simulink model "skarab_fgbe"  (R2018a)
settings: Solver=VariableStepDiscrete  StartTime=0.0  StopTime=50000  RelTol=1e-3
libraries: xbsIndex_r4 x704, casper_library_misc x5, xps_library x3
(part 1 of 9)
settings Model: Creator=cicada  LastModifiedBy=aisaacson
settings SolverCC: ZeroCrossControl=EnableAll
settings DataIOCC: LimitDataPoints=on  SaveFormat=Array  SignalLoggingSaveFormat=ModelDataLogs
settings OptimizationCC: DefaultParameterBehavior=Inlined  ExpressionDepthLimit=2147483647  LifeSpan=inf
settings DebuggingCC: WriteAfterWriteMsg=EnableAllAsError  SignalResolutionControl=TryResolveAllWithWarning  SolverPrmCheckMsg=warning  FcnCallInpInsideContextMsg=warning  AllowSymbolicDim=off  StateNameClashWarn=warning  LibraryContextMissingDiagnostic=warning  StrictBusMsg=ErrorOnBusTreatedAsVector  SFUnexpectedBacktrackingDiag=warning  SFNoUnconditionalDefaultTransitionDiag=warning  SFExecutionAtInitializationDiag=none
settings HardwareCC: ProdBitPerPointer=32  ProdBitPerSizeT=32  ProdBitPerPtrDiffT=32  ProdLargestAtomicFloat=None  ProdIntDivRoundTo=Undefined  ProdEndianess=Unspecified  ProdWordSize=32  ProdHWDeviceType=32-bit Generic
settings ModelReferenceCC: PropagateSignalLabelsOutOfModel=off
settings CodeAppCC: StateflowObjectComments=on
settings GRTTargetCC: TargetLangStandard=C89/C90 (ANSI)  GeneratePreprocessorConditionals=Disable all  CombineOutputUpdateFcns=off  GRTInterface=on
settings ConfigComp: CovMetricSettings=dw  CovHtmlReporting=on  CovSaveCumulativeToWorkspaceVar=on  CovSaveSingleToWorkspaceVar=on  CovExternalEMLEnable=off

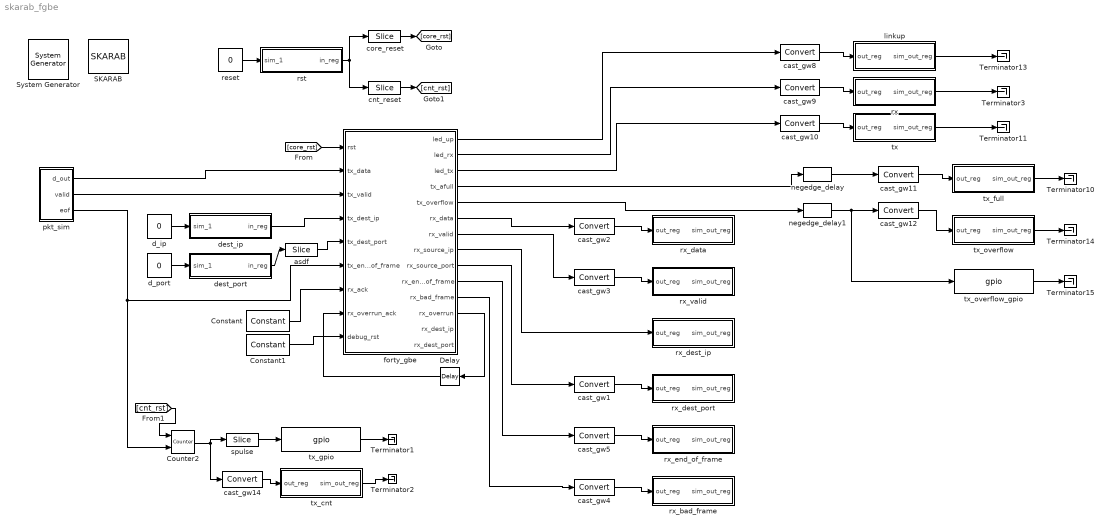
== system skarab_fgbe ==
  " System Generator" : xbsIndex_r4/ System Generator  Tag=genX  xilinxfamily=virtex7  part=xc7vx690t  speed=-2  package=ffg1927  synthesis_tool=XST  clock_wrapper=Clock Enables  directory=/data/casper/mlib_devel_sw_reg_defaults/jasper_library/test_models/skarab_fgbe/sysgen  proj_type=Project Navigator  Synth_file=XST Defaults  Impl_file=ISE Defaults  testbench=off  simulink_period=1  sysclk_period=5.8824  dcm_input_clock_period=10  incr_netlist=off  trim_vbits=Everywhere in SubSystem  dbl_ovrd=According to Block Masks  core_generation=According to Block Masks  run_coregen=off  deprecated_control=off  eval_field=0  block_type=sysgen
      settings: block_version=11.4
  Constant : xbsIndex_r4/Constant  const=1  gui_display_data_type=Boolean  arith_type=Boolean  n_bits=16  bin_pt=14  preci_type=Single  exp_width=8  frac_width=24  explicit_period=on  period=1  equ=P=C  opselect=C  inp2=PCIN>>17  opr=+  inp1=P  carry=CIN  dbl_ovrd=off  block_type=constant
  Constant1 : xbsIndex_r4/Constant  const=0  gui_display_data_type=Boolean  arith_type=Boolean  n_bits=16  bin_pt=14  preci_type=Single  exp_width=8  frac_width=24  explicit_period=on  period=1  equ=P=C  opselect=C  inp2=PCIN>>17  opr=+  inp1=P  carry=CIN  dbl_ovrd=off  block_type=constant
  Counter2 : xbsIndex_r4/Counter  cnt_type=Free Running  cnt_to=Inf  operation=Up  start_count=0  cnt_by_val=1  arith_type=Unsigned  n_bits=32  bin_pt=0  load_pin=off  rst=on  en=on  explicit_period=on  period=1  use_behavioral_HDL=off  implementation=Fabric  dbl_ovrd=off  block_type=counter
      settings: block_version=11.4
  Delay : xbsIndex_r4/Delay  rst=off  infoeditControl=Selection of Reset will increase slice count due to use of real FFs and instead of SRLs  en=off  latency=1  reg_retiming=on  dbl_ovrd=off  block_type=delay
      settings: block_version=11.4
  SKARAB : xps_library/Platforms/SKARAB  Tag=xps:xsg  hw_sys=SKARAB:xc7vx690t  clk_src=sys_clk  clk_rate=170  sample_period=1  synthesis_tool=XST
      settings: SourceProductName=CASPER XPS Blockset
  Terminator{1..3,10..11,13..15} (8 alike) : Terminator
  asdf : xbsIndex_r4/Slice  nbits=16  boolean_output=off  mode=Lower Bit Location + Width  bit1=0  base1=MSB of Input  bit0=0  base0=LSB of Input  dbl_ovrd=off  block_type=slice
  cast_gw{1..5,8..12,14} (11 alike) : xbsIndex_r4/Convert  gui_display_data_type=Fixed-point  arith_type=Unsigned  n_bits=32  bin_pt=0  float_type=Single  exp_bits=8  fraction_bits=24  quantization=Truncate  overflow=Wrap  en=off  latency=0  pipeline=off  dbl_ovrd=off  block_type=convert
  cnt_reset : xbsIndex_r4/Slice  nbits=1  boolean_output=on  mode=Lower Bit Location + Width  bit1=0  base1=MSB of Input  bit0=0  base0=LSB of Input  dbl_ovrd=off  block_type=slice
  core_reset : xbsIndex_r4/Slice  nbits=1  boolean_output=on  mode=Lower Bit Location + Width  bit1=0  base1=MSB of Input  bit0=1  base0=LSB of Input  dbl_ovrd=off  block_type=slice
  d_ip : Constant  Value=0
  d_port : Constant  Value=0
  dest_ip : Subsystem  Tag=xps:sw_reg  AncestorBlock=xps_library/Memory/software_register  mask(swreg){io_dir=From Processor, io_delay=0, init_val=1234, sample_period=1, names=reg, bitwidths=32, bin_pts=0, arith_types=0, sim_port=on, show_format=on}
      mask prompts: io_dir "I/O direction"; io_delay "I/O delay"; init_val "Initial Value"; sample_period "Sample period"; names "Bitfield names [msb...lsb]"; bitwidths "Bitfield widths"; bin_pts "Bitfield binary pts"; arith_types "Bitfield types, ufix=0, fix=1, bool=2"; sim_port "Provide sim input/output?"; show_format "Print format string?"
      mask help: A 32-bit software-accessible register. Can be divided into bitfields of varying widths and types using the fields in the block mask.
      mask init:
      | swreg_init(gcb)
      settings: AttributesFormatString=1input:uf32.0 = 32 bits
      mask TypeOptions io_dir: To Processor | From Processor
      mask Callback io_dir:
      | mask_enables = get_param(gcb, 'MaskEnables');
      | mask_names = get_param(gcb, 'MaskNames');
      | if strcmp(get_param(gcb, 'io_dir'), 'To Processor'),
      |     mask_enables{ismember(mask_names, 'sample_period')} = 'off';
      | else
      |     mask_enables{ismember(mask_names, 'sample_period')} = 'on';
      | end
      | set_param(gcb, 'MaskEnables', mask_enables);
      mask DialogControl ParameterTabVar0 Prompt: Setup
  dest_port : Subsystem  Tag=xps:sw_reg  AncestorBlock=xps_library/Memory/software_register  mask(swreg){io_dir=From Processor, io_delay=0, init_val=64000, sample_period=1, names=reg, bitwidths=32, bin_pts=0, arith_types=0, sim_port=on, show_format=on}
      mask prompts: io_dir "I/O direction"; io_delay "I/O delay"; init_val "Initial Value"; sample_period "Sample period"; names "Bitfield names [msb...lsb]"; bitwidths "Bitfield widths"; bin_pts "Bitfield binary pts"; arith_types "Bitfield types, ufix=0, fix=1, bool=2"; sim_port "Provide sim input/output?"; show_format "Print format string?"
      mask help: A 32-bit software-accessible register. Can be divided into bitfields of varying widths and types using the fields in the block mask.
      mask init:
      | swreg_init(gcb)
      settings: AttributesFormatString=1input:uf32.0 = 32 bits
      mask TypeOptions io_dir: To Processor | From Processor
      mask Callback io_dir:
      | mask_enables = get_param(gcb, 'MaskEnables');
      | mask_names = get_param(gcb, 'MaskNames');
      | if strcmp(get_param(gcb, 'io_dir'), 'To Processor'),
      |     mask_enables{ismember(mask_names, 'sample_period')} = 'off';
      | else
      |     mask_enables{ismember(mask_names, 'sample_period')} = 'on';
      | end
      | set_param(gcb, 'MaskEnables', mask_enables);
      mask DialogControl ParameterTabVar0 Prompt: Setup
  forty_gbe : Subsystem  Tag=xps:forty_gbe  AncestorBlock=xps_library/IO/forty_gbe  mask(forty_gbe){flavour=cx4, slot=1, port_r1=0, port_r2_cx4=0, port_r2_sfpp=0, port=0, rx_dist_ram=on, large_frames=off, input_pipeline_delay=3, show_param=off, pre_emph_r2=0.74, pre_emph=3, post_emph_r2=0.18, rxeqmix_r2=7, swing_r2=940, swing=800, fab_en=on, fab_mac=hex2dec('123456780000'), fab_ip=192*(2^24) + 168*(2^16) + 5*(2^8) + 20*(2^0), fab_udp=10000, fab_gate=1, cpu_rx_en=on, cpu_tx_en=on, ttl=hex2dec('FF'), promisc_mode=off, debug_ctr_width=16, debug_en_all=off, debug_dis_all=off, txctr=off, txerrctr=off, txerrctr_len=100, txofctr=off, txfullctr=off, txvldctr=off, txsnaplen=256, rxctr=off, rxerrctr=off, rxerrctr_len=100, rxofctr=off, rxbadctr=off, rxvldctr=off, rxeofctr=off, rxsnaplen=0 - no snap, rxsrcip=on, rxdstip=on}
      mask prompts: flavour "Mezzanine card flavour"; slot "Card slot"; port_r1 "Port"; port_r2_cx4 "Port"; port_r2_sfpp "Port"; rx_dist_ram "Shallow RX Fifo (Beware overruns!)"; large_frames "Enable Large TX Frames (8k+512)"; input_pipeline_delay "Incoming pipeline delay"; show_param "---------------------- Show Implementation Parameters -----------------------------------------------------------------------------------"; pre_emph_r2 "Pre-emphasis (dB)"; pre_emph "Pre-emphasis"; post_emph_r2 "Post-emphasis (dB)"; rxeqmix_r2 "Receive equalisation"; swing_r2 "Driver Swing Control (mVppd)"; swing "Differential swing"; fab_en "Enable fabric on startup"; fab_mac "Fabric MAC Address"; fab_ip "Fabric IP Address"; fab_udp "Fabric UDP Port"; fab_gate "Fabric Gateway"; cpu_rx_en "Enable CPU RX"; cpu_tx_en "Enable CPU TX"; promisc_mode "Promiscuous mode"; debug_ctr_width "Debug counter width"; debug_en_all "Enable all counters (overrides individual settings)"; debug_dis_all "Disable all counters (overrides individual settings)"; txctr "TX - core_txctr"; txerrctr "TX packet length error - core_txerrctr"; txerrctr_len "-- expected TX packet length"; txofctr "TX overflow - core_txofctr"; txfullctr "TX full - core_txfullctr"; txvldctr "TX valid cycle - core_txvldctr"; txsnaplen "TX snapshot length"; rxctr "RX - core_rxctr"; rxerrctr "RX packet length error - core_rxerrctr"; rxerrctr_len "-- expected RX packet length"; rxofctr "RX overflow - core_rxofctr"; rxbadctr "RX bad - core_rxbadctr"; rxvldctr "RX valid cycle - core_rxvldctr"; rxeofctr "RX eof - core_rxeofctr"; rxsnaplen "RX snapshot length"; rxsrcip "RX snapshot - include source IPs"; rxdstip "RX snapshot - include destination IPs"
      mask help: This block sends and receives UDP frames (packets). It accepts a 64 bit wide data stream with user-determined frame breaks. The data stream is wrapped in a UDP frame for transmission. Incoming UDP packets are unwrapped and the data presented as a 64 bit wide stream.
      mask init:
      | temp = eval(get_param(gcb, 'debug_ctr_width'));
      | if temp <= 0,
      |     error('Debug counters cannot be <= zero.');
      | end
      | forty_gbe_mask(gcb)
      settings: AttributesFormatString=incoming_latency=3
      mask TypeOptions flavour: sfp+ | cx4
      mask Callback flavour: forty_gbe_callback
      mask TypeOptions slot: 0 | 1
      mask TypeOptions port_r1: 0 | 1 | 2 | 3
      mask TypeOptions port_r2_cx4: 0 | 1 | 2
      mask TypeOptions port_r2_sfpp: 0 | 1 | 2 | 3
      mask TypeOptions port: 0 | 1 | 2 | 3
      mask Callback show_param: forty_gbe_callback
      mask TypeOptions pre_emph_r2: 0.15 | 0.3 | 0.45 | 0.61 | 0.74 | 0.91 | 1.07 | 1.25 | 1.36 | 1.55 | 1.74 | 1.94 | 2.11 | 2.32 | 2.54 | 2.77
      mask TypeOptions pre_emph: 0 | 1 | 2 | 3
      mask TypeOptions post_emph_r2: 0.18 | 0.19 | 0.2 | 0.39 | 0.63 | 0.82 | 1.07 | 1.32 | 1.6 | 1.65 | 1.94 | 2.21 | 2.52 | 2.76 | 3.08 | 3.41 | 3.77 | 3.97 | 4.36 | 4.73 | 5.16 | 5.47 | 5.93 | 6.38 | 6.89
      mask TypeOptions rxeqmix_r2: 0 | 1 | 2 | 3 | 4 | 5 | 6 | 7
      mask TypeOptions swing_r2: 110 | 210 | 310 | 400 | 480 | 570 | 660 | 740 | 810 | 880 | 940 | 990 | 1040 | 1080 | 1110 | 1130
      mask TypeOptions swing: 400 | 500 | 600 | 700 | 800
      mask Callback debug_en_all:
      | if strcmp(get_param(gcb, 'debug_en_all'), 'on')
      |     set_param(gcb, 'debug_dis_all', 'off')
      | end
      mask Callback debug_dis_all:
      | if strcmp(get_param(gcb, 'debug_dis_all'), 'on')
      |     set_param(gcb, 'debug_en_all', 'off')
      | end
      mask Callback txerrctr:
      | blk = gcb;
      | mask_visibilities = get_param(blk, 'MaskVisibilities');
      | mask_names = get_param(blk, 'MaskNames');
      | if strcmp(get_param(blk, 'txerrctr'), 'on')
      |     mask_visibilities{ismember(mask_names, 'txerrctr_len')} = 'on';
      | else
      |     mask_visibilities{ismember(mask_names, 'txerrctr_len')} = 'off';
      | end
      | set_param(blk, 'MaskVisibilities', mask_visibilities);
      mask TypeOptions txsnaplen: 0 - no snap | 256 | 512 | 1024 | 2048 | 4096 | 8192 | 16384
      mask Callback rxerrctr:
      | blk = gcb;
      | mask_visibilities = get_param(blk, 'MaskVisibilities');
      | mask_names = get_param(blk, 'MaskNames');
      | if strcmp(get_param(blk, 'rxerrctr'), 'on')
      |     mask_visibilities{ismember(mask_names, 'rxerrctr_len')} = 'on';
      | else
      |     mask_visibilities{ismember(mask_names, 'rxerrctr_len')} = 'off';
      | end
      | set_param(blk, 'MaskVisibilities', mask_visibilities);
      mask TypeOptions rxsnaplen: 0 - no snap | 256 | 512 | 1024 | 2048 | 4096 | 8192 | 16384
      mask DialogControl ParameterTabVar0 Prompt: Core
      mask DialogControl ParameterTabVar01 Prompt: Debug counters
      mask DialogControl Control2 Prompt: -------------------------------------
      mask DialogControl Control2_copy Prompt: -------------------------------------
  linkup : Subsystem  Tag=xps:sw_reg  AncestorBlock=xps_library/Memory/software_register  mask(swreg){io_dir=To Processor, io_delay=0, init_val=0, sample_period=1, names=reg, bitwidths=32, bin_pts=0, arith_types=0, sim_port=on, show_format=on}
      mask prompts: io_dir "I/O direction"; io_delay "I/O delay"; init_val "Initial Value"; sample_period "Sample period"; names "Bitfield names [msb...lsb]"; bitwidths "Bitfield widths"; bin_pts "Bitfield binary pts"; arith_types "Bitfield types, ufix=0, fix=1, bool=2"; sim_port "Provide sim input/output?"; show_format "Print format string?"
      mask help: A 32-bit software-accessible register. Can be divided into bitfields of varying widths and types using the fields in the block mask.
      mask init:
      | swreg_init(gcb)
      settings: AttributesFormatString=1output:uf32.0 = 32 bits
      mask TypeOptions io_dir: To Processor | From Processor
      mask Callback io_dir:
      | mask_enables = get_param(gcb, 'MaskEnables');
      | mask_names = get_param(gcb, 'MaskNames');
      | if strcmp(get_param(gcb, 'io_dir'), 'To Processor'),
      |     mask_enables{ismember(mask_names, 'sample_period')} = 'off';
      | else
      |     mask_enables{ismember(mask_names, 'sample_period')} = 'on';
      | end
      | set_param(gcb, 'MaskEnables', mask_enables);
      mask DialogControl ParameterTabVar0 Prompt: Setup
  negedge_delay : casper_library_misc/negedge_delay  pulse_len=2^20
      settings: SourceProductName=CASPER DSP Blockset
  negedge_delay1 : casper_library_misc/negedge_delay  pulse_len=2^20
      settings: SourceProductName=CASPER DSP Blockset
  pkt_sim : Subsystem
  reset : Constant  Value=0
  rst : Subsystem  Tag=xps:sw_reg  AncestorBlock=xps_library/Memory/software_register  mask(swreg){io_dir=From Processor, io_delay=0, init_val=0, sample_period=1, names=reg, bitwidths=32, bin_pts=0, arith_types=0, sim_port=on, show_format=on}
      mask prompts: io_dir "I/O direction"; io_delay "I/O delay"; init_val "Initial Value"; sample_period "Sample period"; names "Bitfield names [msb...lsb]"; bitwidths "Bitfield widths"; bin_pts "Bitfield binary pts"; arith_types "Bitfield types, ufix=0, fix=1, bool=2"; sim_port "Provide sim input/output?"; show_format "Print format string?"
      mask help: A 32-bit software-accessible register. Can be divided into bitfields of varying widths and types using the fields in the block mask.
      mask init:
      | swreg_init(gcb)
      settings: AttributesFormatString=1input:uf32.0 = 32 bits
      mask TypeOptions io_dir: To Processor | From Processor
      mask Callback io_dir:
      | mask_enables = get_param(gcb, 'MaskEnables');
      | mask_names = get_param(gcb, 'MaskNames');
      | if strcmp(get_param(gcb, 'io_dir'), 'To Processor'),
      |     mask_enables{ismember(mask_names, 'sample_period')} = 'off';
      | else
      |     mask_enables{ismember(mask_names, 'sample_period')} = 'on';
      | end
      | set_param(gcb, 'MaskEnables', mask_enables);
      mask DialogControl ParameterTabVar0 Prompt: Setup
  rx : Subsystem  Tag=xps:sw_reg  AncestorBlock=xps_library/Memory/software_register  mask(swreg){io_dir=To Processor, io_delay=0, init_val=0, sample_period=1, names=reg, bitwidths=32, bin_pts=0, arith_types=0, sim_port=on, show_format=on}
      mask prompts: io_dir "I/O direction"; io_delay "I/O delay"; init_val "Initial Value"; sample_period "Sample period"; names "Bitfield names [msb...lsb]"; bitwidths "Bitfield widths"; bin_pts "Bitfield binary pts"; arith_types "Bitfield types, ufix=0, fix=1, bool=2"; sim_port "Provide sim input/output?"; show_format "Print format string?"
      mask help: A 32-bit software-accessible register. Can be divided into bitfields of varying widths and types using the fields in the block mask.
      mask init:
      | swreg_init(gcb)
      settings: AttributesFormatString=1output:uf32.0 = 32 bits
      mask TypeOptions io_dir: To Processor | From Processor
      mask Callback io_dir:
      | mask_enables = get_param(gcb, 'MaskEnables');
      | mask_names = get_param(gcb, 'MaskNames');
      | if strcmp(get_param(gcb, 'io_dir'), 'To Processor'),
      |     mask_enables{ismember(mask_names, 'sample_period')} = 'off';
      | else
      |     mask_enables{ismember(mask_names, 'sample_period')} = 'on';
      | end
      | set_param(gcb, 'MaskEnables', mask_enables);
      mask DialogControl ParameterTabVar0 Prompt: Setup
  rx_bad_frame : Subsystem  Tag=xps:sw_reg  AncestorBlock=xps_library/Memory/software_register  mask(swreg){io_dir=To Processor, io_delay=0, init_val=0, sample_period=1, names=reg, bitwidths=32, bin_pts=0, arith_types=0, sim_port=on, show_format=on}
      mask prompts: io_dir "I/O direction"; io_delay "I/O delay"; init_val "Initial Value"; sample_period "Sample period"; names "Bitfield names [msb...lsb]"; bitwidths "Bitfield widths"; bin_pts "Bitfield binary pts"; arith_types "Bitfield types, ufix=0, fix=1, bool=2"; sim_port "Provide sim input/output?"; show_format "Print format string?"
      mask help: A 32-bit software-accessible register. Can be divided into bitfields of varying widths and types using the fields in the block mask.
      mask init:
      | swreg_init(gcb)
      settings: AttributesFormatString=1output:uf32.0 = 32 bits
      mask TypeOptions io_dir: To Processor | From Processor
      mask Callback io_dir:
      | mask_enables = get_param(gcb, 'MaskEnables');
      | mask_names = get_param(gcb, 'MaskNames');
      | if strcmp(get_param(gcb, 'io_dir'), 'To Processor'),
      |     mask_enables{ismember(mask_names, 'sample_period')} = 'off';
      | else
      |     mask_enables{ismember(mask_names, 'sample_period')} = 'on';
      | end
      | set_param(gcb, 'MaskEnables', mask_enables);
      mask DialogControl ParameterTabVar0 Prompt: Setup
  rx_data : Subsystem  Tag=xps:sw_reg  AncestorBlock=xps_library/Memory/software_register  mask(swreg){io_dir=To Processor, io_delay=0, init_val=0, sample_period=1, names=reg, bitwidths=32, bin_pts=0, arith_types=0, sim_port=on, show_format=on}
      mask prompts: io_dir "I/O direction"; io_delay "I/O delay"; init_val "Initial Value"; sample_period "Sample period"; names "Bitfield names [msb...lsb]"; bitwidths "Bitfield widths"; bin_pts "Bitfield binary pts"; arith_types "Bitfield types, ufix=0, fix=1, bool=2"; sim_port "Provide sim input/output?"; show_format "Print format string?"
      mask help: A 32-bit software-accessible register. Can be divided into bitfields of varying widths and types using the fields in the block mask.
      mask init:
      | swreg_init(gcb)
      settings: AttributesFormatString=1output:uf32.0 = 32 bits
      mask TypeOptions io_dir: To Processor | From Processor
      mask Callback io_dir:
      | mask_enables = get_param(gcb, 'MaskEnables');
      | mask_names = get_param(gcb, 'MaskNames');
      | if strcmp(get_param(gcb, 'io_dir'), 'To Processor'),
      |     mask_enables{ismember(mask_names, 'sample_period')} = 'off';
      | else
      |     mask_enables{ismember(mask_names, 'sample_period')} = 'on';
      | end
      | set_param(gcb, 'MaskEnables', mask_enables);
      mask DialogControl ParameterTabVar0 Prompt: Setup
  rx_dest_ip : Subsystem  Tag=xps:sw_reg  AncestorBlock=xps_library/Memory/software_register  mask(swreg){io_dir=To Processor, io_delay=0, init_val=0, sample_period=1, names=reg, bitwidths=32, bin_pts=0, arith_types=0, sim_port=on, show_format=on}
      mask prompts: io_dir "I/O direction"; io_delay "I/O delay"; init_val "Initial Value"; sample_period "Sample period"; names "Bitfield names [msb...lsb]"; bitwidths "Bitfield widths"; bin_pts "Bitfield binary pts"; arith_types "Bitfield types, ufix=0, fix=1, bool=2"; sim_port "Provide sim input/output?"; show_format "Print format string?"
      mask help: A 32-bit software-accessible register. Can be divided into bitfields of varying widths and types using the fields in the block mask.
      mask init:
      | swreg_init(gcb)
      settings: AttributesFormatString=1output:uf32.0 = 32 bits
      mask TypeOptions io_dir: To Processor | From Processor
      mask Callback io_dir:
      | mask_enables = get_param(gcb, 'MaskEnables');
      | mask_names = get_param(gcb, 'MaskNames');
      | if strcmp(get_param(gcb, 'io_dir'), 'To Processor'),
      |     mask_enables{ismember(mask_names, 'sample_period')} = 'off';
      | else
      |     mask_enables{ismember(mask_names, 'sample_period')} = 'on';
      | end
      | set_param(gcb, 'MaskEnables', mask_enables);
      mask DialogControl ParameterTabVar0 Prompt: Setup
  rx_dest_port : Subsystem  Tag=xps:sw_reg  AncestorBlock=xps_library/Memory/software_register  mask(swreg){io_dir=To Processor, io_delay=0, init_val=0, sample_period=1, names=reg, bitwidths=32, bin_pts=0, arith_types=0, sim_port=on, show_format=on}
      mask prompts: io_dir "I/O direction"; io_delay "I/O delay"; init_val "Initial Value"; sample_period "Sample period"; names "Bitfield names [msb...lsb]"; bitwidths "Bitfield widths"; bin_pts "Bitfield binary pts"; arith_types "Bitfield types, ufix=0, fix=1, bool=2"; sim_port "Provide sim input/output?"; show_format "Print format string?"
      mask help: A 32-bit software-accessible register. Can be divided into bitfields of varying widths and types using the fields in the block mask.
      mask init:
      | swreg_init(gcb)
      settings: AttributesFormatString=1output:uf32.0 = 32 bits
      mask TypeOptions io_dir: To Processor | From Processor
      mask Callback io_dir:
      | mask_enables = get_param(gcb, 'MaskEnables');
      | mask_names = get_param(gcb, 'MaskNames');
      | if strcmp(get_param(gcb, 'io_dir'), 'To Processor'),
      |     mask_enables{ismember(mask_names, 'sample_period')} = 'off';
      | else
      |     mask_enables{ismember(mask_names, 'sample_period')} = 'on';
      | end
      | set_param(gcb, 'MaskEnables', mask_enables);
      mask DialogControl ParameterTabVar0 Prompt: Setup
  rx_end_of_frame : Subsystem  Tag=xps:sw_reg  AncestorBlock=xps_library/Memory/software_register  mask(swreg){io_dir=To Processor, io_delay=0, init_val=0, sample_period=1, names=reg, bitwidths=32, bin_pts=0, arith_types=0, sim_port=on, show_format=on}
      mask prompts: io_dir "I/O direction"; io_delay "I/O delay"; init_val "Initial Value"; sample_period "Sample period"; names "Bitfield names [msb...lsb]"; bitwidths "Bitfield widths"; bin_pts "Bitfield binary pts"; arith_types "Bitfield types, ufix=0, fix=1, bool=2"; sim_port "Provide sim input/output?"; show_format "Print format string?"
      mask help: A 32-bit software-accessible register. Can be divided into bitfields of varying widths and types using the fields in the block mask.
      mask init:
      | swreg_init(gcb)
      settings: AttributesFormatString=1output:uf32.0 = 32 bits
      mask TypeOptions io_dir: To Processor | From Processor
      mask Callback io_dir:
      | mask_enables = get_param(gcb, 'MaskEnables');
      | mask_names = get_param(gcb, 'MaskNames');
      | if strcmp(get_param(gcb, 'io_dir'), 'To Processor'),
      |     mask_enables{ismember(mask_names, 'sample_period')} = 'off';
      | else
      |     mask_enables{ismember(mask_names, 'sample_period')} = 'on';
      | end
      | set_param(gcb, 'MaskEnables', mask_enables);
      mask DialogControl ParameterTabVar0 Prompt: Setup
  rx_valid : Subsystem  Tag=xps:sw_reg  AncestorBlock=xps_library/Memory/software_register  mask(swreg){io_dir=To Processor, io_delay=0, init_val=0, sample_period=1, names=reg, bitwidths=32, bin_pts=0, arith_types=0, sim_port=on, show_format=on}
      mask prompts: io_dir "I/O direction"; io_delay "I/O delay"; init_val "Initial Value"; sample_period "Sample period"; names "Bitfield names [msb...lsb]"; bitwidths "Bitfield widths"; bin_pts "Bitfield binary pts"; arith_types "Bitfield types, ufix=0, fix=1, bool=2"; sim_port "Provide sim input/output?"; show_format "Print format string?"
      mask help: A 32-bit software-accessible register. Can be divided into bitfields of varying widths and types using the fields in the block mask.
      mask init:
      | swreg_init(gcb)
      settings: AttributesFormatString=1output:uf32.0 = 32 bits
      mask TypeOptions io_dir: To Processor | From Processor
      mask Callback io_dir:
      | mask_enables = get_param(gcb, 'MaskEnables');
      | mask_names = get_param(gcb, 'MaskNames');
      | if strcmp(get_param(gcb, 'io_dir'), 'To Processor'),
      |     mask_enables{ismember(mask_names, 'sample_period')} = 'off';
      | else
      |     mask_enables{ismember(mask_names, 'sample_period')} = 'on';
      | end
      | set_param(gcb, 'MaskEnables', mask_enables);
      mask DialogControl ParameterTabVar0 Prompt: Setup
  spulse : xbsIndex_r4/Slice  nbits=1  boolean_output=on  mode=Lower Bit Location + Width  bit1=0  base1=MSB of Input  bit0=27-12  base0=LSB of Input  dbl_ovrd=off  block_type=slice
  tx : Subsystem  Tag=xps:sw_reg  AncestorBlock=xps_library/Memory/software_register  mask(swreg){io_dir=To Processor, io_delay=0, init_val=0, sample_period=1, names=reg, bitwidths=32, bin_pts=0, arith_types=0, sim_port=on, show_format=on}
      mask prompts: io_dir "I/O direction"; io_delay "I/O delay"; init_val "Initial Value"; sample_period "Sample period"; names "Bitfield names [msb...lsb]"; bitwidths "Bitfield widths"; bin_pts "Bitfield binary pts"; arith_types "Bitfield types, ufix=0, fix=1, bool=2"; sim_port "Provide sim input/output?"; show_format "Print format string?"
      mask help: A 32-bit software-accessible register. Can be divided into bitfields of varying widths and types using the fields in the block mask.
      mask init:
      | swreg_init(gcb)
      settings: AttributesFormatString=1output:uf32.0 = 32 bits
      mask TypeOptions io_dir: To Processor | From Processor
      mask Callback io_dir:
      | mask_enables = get_param(gcb, 'MaskEnables');
      | mask_names = get_param(gcb, 'MaskNames');
      | if strcmp(get_param(gcb, 'io_dir'), 'To Processor'),
      |     mask_enables{ismember(mask_names, 'sample_period')} = 'off';
      | else
      |     mask_enables{ismember(mask_names, 'sample_period')} = 'on';
      | end
      | set_param(gcb, 'MaskEnables', mask_enables);
      mask DialogControl ParameterTabVar0 Prompt: Setup
  tx_cnt : Subsystem  Tag=xps:sw_reg  AncestorBlock=xps_library/Memory/software_register  mask(swreg){io_dir=To Processor, io_delay=0, init_val=0, sample_period=1, names=reg, bitwidths=32, bin_pts=0, arith_types=0, sim_port=on, show_format=on}
      mask prompts: io_dir "I/O direction"; io_delay "I/O delay"; init_val "Initial Value"; sample_period "Sample period"; names "Bitfield names [msb...lsb]"; bitwidths "Bitfield widths"; bin_pts "Bitfield binary pts"; arith_types "Bitfield types, ufix=0, fix=1, bool=2"; sim_port "Provide sim input/output?"; show_format "Print format string?"
      mask help: A 32-bit software-accessible register. Can be divided into bitfields of varying widths and types using the fields in the block mask.
      mask init:
      | swreg_init(gcb)
      settings: AttributesFormatString=1output:uf32.0 = 32 bits
      mask TypeOptions io_dir: To Processor | From Processor
      mask Callback io_dir:
      | mask_enables = get_param(gcb, 'MaskEnables');
      | mask_names = get_param(gcb, 'MaskNames');
      | if strcmp(get_param(gcb, 'io_dir'), 'To Processor'),
      |     mask_enables{ismember(mask_names, 'sample_period')} = 'off';
      | else
      |     mask_enables{ismember(mask_names, 'sample_period')} = 'on';
      | end
      | set_param(gcb, 'MaskEnables', mask_enables);
      mask DialogControl ParameterTabVar0 Prompt: Setup
  tx_full : Subsystem  Tag=xps:sw_reg  AncestorBlock=xps_library/Memory/software_register  mask(swreg){io_dir=To Processor, io_delay=0, init_val=0, sample_period=1, names=reg, bitwidths=32, bin_pts=0, arith_types=0, sim_port=on, show_format=on}
      mask prompts: io_dir "I/O direction"; io_delay "I/O delay"; init_val "Initial Value"; sample_period "Sample period"; names "Bitfield names [msb...lsb]"; bitwidths "Bitfield widths"; bin_pts "Bitfield binary pts"; arith_types "Bitfield types, ufix=0, fix=1, bool=2"; sim_port "Provide sim input/output?"; show_format "Print format string?"
      mask help: A 32-bit software-accessible register. Can be divided into bitfields of varying widths and types using the fields in the block mask.
      mask init:
      | swreg_init(gcb)
      settings: AttributesFormatString=1output:uf32.0 = 32 bits
      mask TypeOptions io_dir: To Processor | From Processor
      mask Callback io_dir:
      | mask_enables = get_param(gcb, 'MaskEnables');
      | mask_names = get_param(gcb, 'MaskNames');
      | if strcmp(get_param(gcb, 'io_dir'), 'To Processor'),
      |     mask_enables{ismember(mask_names, 'sample_period')} = 'off';
      | else
      |     mask_enables{ismember(mask_names, 'sample_period')} = 'on';
      | end
      | set_param(gcb, 'MaskEnables', mask_enables);
      mask DialogControl ParameterTabVar0 Prompt: Setup
  tx_gpio : xps_library/IO/gpio  Tag=xps:gpio  io_group_params_forwarded=on  io_group=ROACH:led  io_group_real=led  io_group_custom=0  io_dir=out  arith_type=Boolean  bitwidth=1  bin_pt=0  bit_index=0  sample_period=1  use_single_ended=off  use_ddr=off  reg_iob=on  reg_clk_phase=0  termination=None
      settings: SourceProductName=CASPER XPS Blockset
  tx_overflow : Subsystem  Tag=xps:sw_reg  AncestorBlock=xps_library/Memory/software_register  mask(swreg){io_dir=To Processor, io_delay=0, init_val=0, sample_period=1, names=reg, bitwidths=32, bin_pts=0, arith_types=0, sim_port=on, show_format=on}
      mask prompts: io_dir "I/O direction"; io_delay "I/O delay"; init_val "Initial Value"; sample_period "Sample period"; names "Bitfield names [msb...lsb]"; bitwidths "Bitfield widths"; bin_pts "Bitfield binary pts"; arith_types "Bitfield types, ufix=0, fix=1, bool=2"; sim_port "Provide sim input/output?"; show_format "Print format string?"
      mask help: A 32-bit software-accessible register. Can be divided into bitfields of varying widths and types using the fields in the block mask.
      mask init:
      | swreg_init(gcb)
      settings: AttributesFormatString=1output:uf32.0 = 32 bits
      mask TypeOptions io_dir: To Processor | From Processor
      mask Callback io_dir:
      | mask_enables = get_param(gcb, 'MaskEnables');
      | mask_names = get_param(gcb, 'MaskNames');
      | if strcmp(get_param(gcb, 'io_dir'), 'To Processor'),
      |     mask_enables{ismember(mask_names, 'sample_period')} = 'off';
      | else
      |     mask_enables{ismember(mask_names, 'sample_period')} = 'on';
      | end
      | set_param(gcb, 'MaskEnables', mask_enables);
      mask DialogControl ParameterTabVar0 Prompt: Setup
  tx_overflow_gpio : xps_library/IO/gpio  Tag=xps:gpio  io_group_params_forwarded=on  io_group=ROACH:led  io_group_real=led  io_group_custom=0  io_dir=out  arith_type=Boolean  bitwidth=1  bin_pt=0  bit_index=1  sample_period=1  use_single_ended=off  use_ddr=off  reg_iob=on  reg_clk_phase=0  termination=None
      settings: SourceProductName=CASPER XPS Blockset
  wires:
  reset/1 -> rst/1(sim_1)
  rst/1(in_reg) -> core_reset/1, cnt_reset/1
  cnt_reset/1 -> [cnt_rst]
  core_reset/1 -> [core_rst]
  dest_port/1(in_reg) -> asdf/1
  d_ip/1 -> dest_ip/1(sim_1)
  d_port/1 -> dest_port/1(sim_1)
  [core_rst] -> forty_gbe/1(rst)
  pkt_sim/1(d_out) -> forty_gbe/2(tx_data)
  forty_gbe/12(rx_overrun) -> Delay/1
  forty_gbe/1(led_up) -> cast_gw8/1
  forty_gbe/2(led_rx) -> cast_gw9/1
  forty_gbe/3(led_tx) -> cast_gw10/1
  forty_gbe/4(tx_afull) -> negedge_delay/1
  forty_gbe/5(tx_overflow) -> negedge_delay1/1
  Delay/1 -> forty_gbe/8(rx_overrun_ack)
  spulse/1 -> tx_gpio/1
  Counter2/1 -> spulse/1, cast_gw14/1
  [cnt_rst] -> Counter2/1
  tx_gpio/1 -> Terminator1/1
  tx_cnt/1(sim_out_reg) -> Terminator2/1
  tx/1(sim_out_reg) -> Terminator11/1
  tx_full/1(sim_out_reg) -> Terminator10/1
  tx_overflow/1(sim_out_reg) -> Terminator14/1
  tx_overflow_gpio/1 -> Terminator15/1
  negedge_delay/1 -> cast_gw11/1
  pkt_sim/3(eof) -> forty_gbe/6(tx_end_of_frame), Counter2/2
  pkt_sim/2(valid) -> forty_gbe/3(tx_valid)
  cast_gw9/1 -> rx/1(out_reg)
  cast_gw10/1 -> tx/1(out_reg)
  cast_gw11/1 -> tx_full/1(out_reg)
  cast_gw12/1 -> tx_overflow/1(out_reg)
  negedge_delay1/1 -> tx_overflow_gpio/1, cast_gw12/1
  cast_gw14/1 -> tx_cnt/1(out_reg)
  dest_ip/1(in_reg) -> forty_gbe/4(tx_dest_ip)
  asdf/1 -> forty_gbe/5(tx_dest_port)
  Constant/1 -> forty_gbe/7(rx_ack)
  Constant1/1 -> forty_gbe/9(debug_rst)
  forty_gbe/8(rx_source_ip) -> rx_dest_ip/1(out_reg)
  cast_gw1/1 -> rx_dest_port/1(out_reg)
  forty_gbe/9(rx_source_port) -> cast_gw1/1
  forty_gbe/7(rx_valid) -> cast_gw3/1
  forty_gbe/6(rx_data) -> cast_gw2/1
  cast_gw2/1 -> rx_data/1(out_reg)
  cast_gw3/1 -> rx_valid/1(out_reg)
  cast_gw4/1 -> rx_bad_frame/1(out_reg)
  forty_gbe/11(rx_bad_frame) -> cast_gw4/1
  forty_gbe/10(rx_end_of_frame) -> cast_gw5/1
  cast_gw5/1 -> rx_end_of_frame/1(out_reg)
  cast_gw8/1 -> linkup/1(out_reg)
  linkup/1(sim_out_reg) -> Terminator13/1
  rx/1(sim_out_reg) -> Terminator3/1

== system skarab_fgbe/dest_ip ==
  sim_1 : Inport
  convert1_1 : DataTypeConversion  OutDataTypeStr=fixdt('ufix32_En0')  LockScale=on
  convert2_1 : DataTypeConversion  OutDataTypeStr=fixdt('ufix32_En0')  ConvertRealWorld=Stored Integer (SI)  LockScale=on
  gain_1 : Gain
  io_delay : xbsIndex_r4/Delay  rst=off  infoeditControl=Selection of Reset will increase slice count due to use of real FFs and instead of SRLs  en=off  latency=0  reg_retiming=on  dbl_ovrd=off  block_type=delay
  reint1 : xbsIndex_r4/Reinterpret  force_arith_type=on  arith_type=Unsigned  force_bin_pt=on  bin_pt=0  block_type=reinterpret
  skarab_fgbe_dest_ip_user_data_out : xbsIndex_r4/Gateway In  gui_display_data_type=Fixed-point  arith_type=Unsigned  n_bits=32  bin_pt=0  preci_type=Single  exp_width=8  frac_width=24  rows=1  columns=1  quantization="Round  (unbiased: +/- Inf)"  overflow=Saturate  period=1  UseAsADC=off  ADCChannel='1'  interface=None  automatic_assignment=on  address_offset=hex2dec('00')  intf_name=''  intf_description=''  default_value=0  timing_constraint=None  locs_specified=off  LOCs={}  io_standard={}  inherit_from_input=off  hdl_port=on  dbl_ovrd=off  block_type=gatewayin
  slice_reg : xbsIndex_r4/Slice  nbits=32  boolean_output=off  mode=Lower Bit Location + Width  bit1=0  base1=MSB of Input  bit0=0  base0=LSB of Input  dbl_ovrd=off  block_type=slice
  in_reg : Outport
  wires:
  skarab_fgbe_dest_ip_user_data_out/1 -> io_delay/1
  sim_1/1 -> convert1_1/1
  convert1_1/1 -> convert2_1/1
  convert2_1/1 -> gain_1/1
  gain_1/1 -> skarab_fgbe_dest_ip_user_data_out/1
  io_delay/1 -> slice_reg/1
  slice_reg/1 -> reint1/1
  reint1/1 -> in_reg/1

== system skarab_fgbe/dest_port ==
  sim_1 : Inport
  convert1_1 : DataTypeConversion  OutDataTypeStr=fixdt('ufix32_En0')  LockScale=on
  convert2_1 : DataTypeConversion  OutDataTypeStr=fixdt('ufix32_En0')  ConvertRealWorld=Stored Integer (SI)  LockScale=on
  gain_1 : Gain
  io_delay : xbsIndex_r4/Delay  rst=off  infoeditControl=Selection of Reset will increase slice count due to use of real FFs and instead of SRLs  en=off  latency=0  reg_retiming=on  dbl_ovrd=off  block_type=delay
  reint1 : xbsIndex_r4/Reinterpret  force_arith_type=on  arith_type=Unsigned  force_bin_pt=on  bin_pt=0  block_type=reinterpret
  skarab_fgbe_dest_port_user_data_out : xbsIndex_r4/Gateway In  gui_display_data_type=Fixed-point  arith_type=Unsigned  n_bits=32  bin_pt=0  preci_type=Single  exp_width=8  frac_width=24  rows=1  columns=1  quantization="Round  (unbiased: +/- Inf)"  overflow=Saturate  period=1  UseAsADC=off  ADCChannel='1'  interface=None  automatic_assignment=on  address_offset=hex2dec('00')  intf_name=''  intf_description=''  default_value=0  timing_constraint=None  locs_specified=off  LOCs={}  io_standard={}  inherit_from_input=off  hdl_port=on  dbl_ovrd=off  block_type=gatewayin
  slice_reg : xbsIndex_r4/Slice  nbits=32  boolean_output=off  mode=Lower Bit Location + Width  bit1=0  base1=MSB of Input  bit0=0  base0=LSB of Input  dbl_ovrd=off  block_type=slice
  in_reg : Outport
  wires:
  skarab_fgbe_dest_port_user_data_out/1 -> io_delay/1
  sim_1/1 -> convert1_1/1
  convert1_1/1 -> convert2_1/1
  convert2_1/1 -> gain_1/1
  gain_1/1 -> skarab_fgbe_dest_port_user_data_out/1
  io_delay/1 -> slice_reg/1
  slice_reg/1 -> reint1/1
  reint1/1 -> in_reg/1
